simulink model "lab2simulink_2"  (R2024b)
settings: Solver=VariableStepAuto  StartTime=0.0  StopTime=10.0  RelTol=1e-3
undefined symbols (not defined in the file or in its folder): dspblkCoreblockFVToolHelper, gcbh
settings Model: Creator=ttkim2  LastModifiedBy=ttkim2

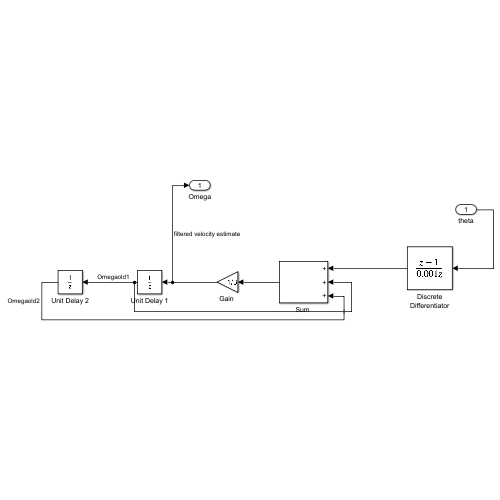
[thumbnail: Simulink's stored preview of the top-level diagram]
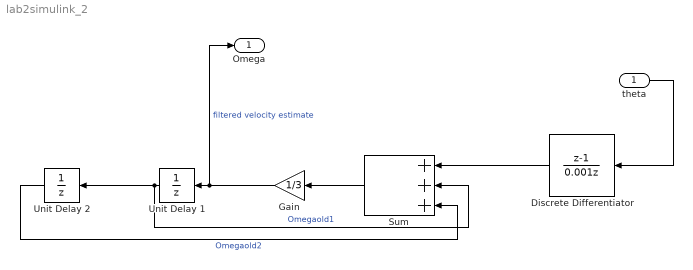
== system lab2simulink_2 ==
  theta : Inport
  Discrete Differentiator : DiscreteTransferFcn  LoadFcn=dspblkCoreblockFVToolHelper(gcbh,'load');  Numerator=[1 -1]  Denominator=[0.001 0]
      settings: CopyFcn=dspblkCoreblockFVToolHelper(gcbh,'copy');  DeleteFcn=dspblkCoreblockFVToolHelper(gcbh,'close');  ModelCloseFcn=dspblkCoreblockFVToolHelper(gcbh,'close');  PreSaveFcn=dspblkCoreblockFVToolHelper(gcbh,'presave');  PostSaveFcn=dspblkCoreblockFVToolHelper(gcbh,'postsave');  CloseFcn=dspblkCoreblockFVToolHelper(gcbh,'close');
  "Gain " : Gain  Gain=1/3
  "Sum " : Sum  Inputs=+++
  Unit Delay 1 : UnitDelay  SampleTime=0.001  HasFrameUpgradeWarning=on
  Unit Delay 2 : UnitDelay  SampleTime=0.001  HasFrameUpgradeWarning=on
  Omega : Outport
  wires:
  Unit Delay 2/1 -> "Sum "/3  "Omegaold2"
  Discrete Differentiator/1 -> "Sum "/1
  Unit Delay 1/1 -> "Sum "/2, Unit Delay 2/1  "Omegaold1"
  "Sum "/1 -> "Gain "/1
  "Gain "/1 -> Omega/1, Unit Delay 1/1  "filtered velocity estimate"
  theta/1 -> Discrete Differentiator/1
